simulink model "rfsoc4x2_ospfb_128"  (R2021a)
settings: Solver=VariableStepAuto  StartTime=0.0  StopTime=2048  RelTol=1e-3
undefined symbols (not defined in the file): pfb_coeff_gen_calc
libraries: xbsIndex_r4 x25898, casper_library_delays x113, casper_library_misc x68, xps_library x1
(part 15 of 221)

== system rfsoc4x2_ospfb_128/rfdc ==
  m00_axis_tdata_sim : Inport
  m02_axis_tdata_sim : Inport  Port=2
  m10_axis_tdata_sim : Inport  Port=3
  m12_axis_tdata_sim : Inport  Port=4
  m20_axis_tdata_sim : Inport  Port=5
  m22_axis_tdata_sim : Inport  Port=6
  m30_axis_tdata_sim : Inport  Port=7
  m32_axis_tdata_sim : Inport  Port=8
  rfsoc4x2_ospfb_128_rfdc_m00_axis_tdata : xbsIndex_r4/Gateway In  gui_display_data_type=Fixed-point  arith_type="Signed  (2's comp)"  n_bits=128  bin_pt=0  preci_type=Single  exp_width=8  frac_width=24  rows=1  columns=1  quantization="Round  (unbiased: +/- Inf)"  overflow=Saturate  period=1  UseAsADC=off  ADCChannel='1'  interface=None  automatic_assignment=on  address_offset=hex2dec('00')  intf_name=''  intf_description=''  default_value=0  timing_constraint=None  locs_specified=off  LOCs={}  io_standard={}  inherit_from_input=off  hdl_port=on  dbl_ovrd=off  block_type=gatewayin
  rfsoc4x2_ospfb_128_rfdc_m02_axis_tdata : xbsIndex_r4/Gateway In  gui_display_data_type=Fixed-point  arith_type="Signed  (2's comp)"  n_bits=128  bin_pt=0  preci_type=Single  exp_width=8  frac_width=24  rows=1  columns=1  quantization="Round  (unbiased: +/- Inf)"  overflow=Saturate  period=1  UseAsADC=off  ADCChannel='1'  interface=None  automatic_assignment=on  address_offset=hex2dec('00')  intf_name=''  intf_description=''  default_value=0  timing_constraint=None  locs_specified=off  LOCs={}  io_standard={}  inherit_from_input=off  hdl_port=on  dbl_ovrd=off  block_type=gatewayin
  rfsoc4x2_ospfb_128_rfdc_m10_axis_tdata : xbsIndex_r4/Gateway In  gui_display_data_type=Fixed-point  arith_type="Signed  (2's comp)"  n_bits=128  bin_pt=0  preci_type=Single  exp_width=8  frac_width=24  rows=1  columns=1  quantization="Round  (unbiased: +/- Inf)"  overflow=Saturate  period=1  UseAsADC=off  ADCChannel='1'  interface=None  automatic_assignment=on  address_offset=hex2dec('00')  intf_name=''  intf_description=''  default_value=0  timing_constraint=None  locs_specified=off  LOCs={}  io_standard={}  inherit_from_input=off  hdl_port=on  dbl_ovrd=off  block_type=gatewayin
  rfsoc4x2_ospfb_128_rfdc_m12_axis_tdata : xbsIndex_r4/Gateway In  gui_display_data_type=Fixed-point  arith_type="Signed  (2's comp)"  n_bits=128  bin_pt=0  preci_type=Single  exp_width=8  frac_width=24  rows=1  columns=1  quantization="Round  (unbiased: +/- Inf)"  overflow=Saturate  period=1  UseAsADC=off  ADCChannel='1'  interface=None  automatic_assignment=on  address_offset=hex2dec('00')  intf_name=''  intf_description=''  default_value=0  timing_constraint=None  locs_specified=off  LOCs={}  io_standard={}  inherit_from_input=off  hdl_port=on  dbl_ovrd=off  block_type=gatewayin
  rfsoc4x2_ospfb_128_rfdc_m20_axis_tdata : xbsIndex_r4/Gateway In  gui_display_data_type=Fixed-point  arith_type="Signed  (2's comp)"  n_bits=128  bin_pt=0  preci_type=Single  exp_width=8  frac_width=24  rows=1  columns=1  quantization="Round  (unbiased: +/- Inf)"  overflow=Saturate  period=1  UseAsADC=off  ADCChannel='1'  interface=None  automatic_assignment=on  address_offset=hex2dec('00')  intf_name=''  intf_description=''  default_value=0  timing_constraint=None  locs_specified=off  LOCs={}  io_standard={}  inherit_from_input=off  hdl_port=on  dbl_ovrd=off  block_type=gatewayin
  rfsoc4x2_ospfb_128_rfdc_m22_axis_tdata : xbsIndex_r4/Gateway In  gui_display_data_type=Fixed-point  arith_type="Signed  (2's comp)"  n_bits=128  bin_pt=0  preci_type=Single  exp_width=8  frac_width=24  rows=1  columns=1  quantization="Round  (unbiased: +/- Inf)"  overflow=Saturate  period=1  UseAsADC=off  ADCChannel='1'  interface=None  automatic_assignment=on  address_offset=hex2dec('00')  intf_name=''  intf_description=''  default_value=0  timing_constraint=None  locs_specified=off  LOCs={}  io_standard={}  inherit_from_input=off  hdl_port=on  dbl_ovrd=off  block_type=gatewayin
  rfsoc4x2_ospfb_128_rfdc_m30_axis_tdata : xbsIndex_r4/Gateway In  gui_display_data_type=Fixed-point  arith_type="Signed  (2's comp)"  n_bits=128  bin_pt=0  preci_type=Single  exp_width=8  frac_width=24  rows=1  columns=1  quantization="Round  (unbiased: +/- Inf)"  overflow=Saturate  period=1  UseAsADC=off  ADCChannel='1'  interface=None  automatic_assignment=on  address_offset=hex2dec('00')  intf_name=''  intf_description=''  default_value=0  timing_constraint=None  locs_specified=off  LOCs={}  io_standard={}  inherit_from_input=off  hdl_port=on  dbl_ovrd=off  block_type=gatewayin
  rfsoc4x2_ospfb_128_rfdc_m32_axis_tdata : xbsIndex_r4/Gateway In  gui_display_data_type=Fixed-point  arith_type="Signed  (2's comp)"  n_bits=128  bin_pt=0  preci_type=Single  exp_width=8  frac_width=24  rows=1  columns=1  quantization="Round  (unbiased: +/- Inf)"  overflow=Saturate  period=1  UseAsADC=off  ADCChannel='1'  interface=None  automatic_assignment=on  address_offset=hex2dec('00')  intf_name=''  intf_description=''  default_value=0  timing_constraint=None  locs_specified=off  LOCs={}  io_standard={}  inherit_from_input=off  hdl_port=on  dbl_ovrd=off  block_type=gatewayin
  m00_axis_tdata : Outport
  m02_axis_tdata : Outport  Port=2
  m10_axis_tdata : Outport  Port=3
  m12_axis_tdata : Outport  Port=4
  m20_axis_tdata : Outport  Port=5
  m22_axis_tdata : Outport  Port=6
  m30_axis_tdata : Outport  Port=7
  m32_axis_tdata : Outport  Port=8
  wires:
  m00_axis_tdata_sim/1 -> rfsoc4x2_ospfb_128_rfdc_m00_axis_tdata/1
  rfsoc4x2_ospfb_128_rfdc_m00_axis_tdata/1 -> m00_axis_tdata/1  "m00_axis_tdata"
  m02_axis_tdata_sim/1 -> rfsoc4x2_ospfb_128_rfdc_m02_axis_tdata/1
  rfsoc4x2_ospfb_128_rfdc_m02_axis_tdata/1 -> m02_axis_tdata/1  "m02_axis_tdata"
  m10_axis_tdata_sim/1 -> rfsoc4x2_ospfb_128_rfdc_m10_axis_tdata/1
  rfsoc4x2_ospfb_128_rfdc_m10_axis_tdata/1 -> m10_axis_tdata/1  "m10_axis_tdata"
  m12_axis_tdata_sim/1 -> rfsoc4x2_ospfb_128_rfdc_m12_axis_tdata/1
  rfsoc4x2_ospfb_128_rfdc_m12_axis_tdata/1 -> m12_axis_tdata/1  "m12_axis_tdata"
  m20_axis_tdata_sim/1 -> rfsoc4x2_ospfb_128_rfdc_m20_axis_tdata/1
  rfsoc4x2_ospfb_128_rfdc_m20_axis_tdata/1 -> m20_axis_tdata/1  "m20_axis_tdata"
  m22_axis_tdata_sim/1 -> rfsoc4x2_ospfb_128_rfdc_m22_axis_tdata/1
  rfsoc4x2_ospfb_128_rfdc_m22_axis_tdata/1 -> m22_axis_tdata/1  "m22_axis_tdata"
  m30_axis_tdata_sim/1 -> rfsoc4x2_ospfb_128_rfdc_m30_axis_tdata/1
  rfsoc4x2_ospfb_128_rfdc_m30_axis_tdata/1 -> m30_axis_tdata/1  "m30_axis_tdata"
  m32_axis_tdata_sim/1 -> rfsoc4x2_ospfb_128_rfdc_m32_axis_tdata/1
  rfsoc4x2_ospfb_128_rfdc_m32_axis_tdata/1 -> m32_axis_tdata/1  "m32_axis_tdata"

== system rfsoc4x2_ospfb_128/simple_bram_vacc10 ==
  new_acc : Inport
  din : Inport  Port=2
  Adder : xbsIndex_r4/AddSub  mode=Addition  use_carryin=off  use_carryout=off  en=off  latency=2  precision=User Defined  arith_type=Unsigned  n_bits=n_bits  bin_pt=bin_pt  quantization=Truncate  overflow=Wrap  use_behavioral_HDL=on  hw_selection=Fabric  pipelined=off  use_rpm=on  dbl_ovrd=off  block_type=addsub
      settings: xl_area=[0, 0, 0, 0, 0, 0, 0]  block_version=10.1.3
  Constant : xbsIndex_r4/Constant  const=0  gui_display_data_type=Fixed-point  arith_type=Unsigned  n_bits=n_bits  bin_pt=bin_pt  preci_type=Single  exp_width=8  frac_width=24  explicit_period=on  period=1  equ=P=C  opselect=C  inp2=PCIN>>17  opr=+  inp1=P  carry=CIN  dbl_ovrd=off  block_type=constant
  Mux : xbsIndex_r4/Mux  inputs=2  en=off  latency=0  precision=Full  arith_type="Signed  (2's comp)"  n_bits=8  bin_pt=2  quantization=Truncate  overflow=Wrap  dbl_ovrd=off  block_type=mux
      settings: xl_area=[0, 0, 0, 0, 0, 0, 0]
  delay_bram : Subsystem  mask(delay_bram){DelayLen=vec_len - 2, bram_latency=2}
      mask prompts: DelayLen "Delay By:"; bram_latency "BRAM Latency"
      mask help: A delay block that uses BRAM for its storage.
      mask init:
      | if (DelayLen <= bram_latency)
      | 	error('delay value must be greater than BRAM Latency');
      | end
      | BitWidth = max(ceil(log2(DelayLen)), 2);
      mask Help: eval('xlWeb(''http://casper.berkeley.edu/wiki/Delay_bram'')')
  pulse_ext : Subsystem  mask(pulse_ext){pulse_len=vec_len}
      mask prompts: pulse_len "Length of Pulse"
      mask help:
      | Extends a boolean signal to be high for the specified number of clocks after
      | the last high input.
      mask init:
      | bits = ceil(log2(pulse_len+1));
      mask Help: eval('xlWeb(''http://casper.berkeley.edu/wiki/Pulse_ext'')')
  dout : Outport  VectorParamsAs1DForOutWhenUnconnected=off
  valid : Outport  Port=2  VectorParamsAs1DForOutWhenUnconnected=off
  wires:
  Adder/1 -> delay_bram/1(In1)
  delay_bram/1(Out1) -> dout/1, Mux/2
  new_acc/1 -> pulse_ext/1(in)
  din/1 -> Adder/1
  pulse_ext/1(out) -> valid/1, Mux/1
  Mux/1 -> Adder/2
  Constant/1 -> Mux/3

== system rfsoc4x2_ospfb_128/simple_bram_vacc11 ==
  new_acc : Inport
  din : Inport  Port=2
  Adder : xbsIndex_r4/AddSub  mode=Addition  use_carryin=off  use_carryout=off  en=off  latency=2  precision=User Defined  arith_type=Unsigned  n_bits=n_bits  bin_pt=bin_pt  quantization=Truncate  overflow=Wrap  use_behavioral_HDL=on  hw_selection=Fabric  pipelined=off  use_rpm=on  dbl_ovrd=off  block_type=addsub
      settings: xl_area=[0, 0, 0, 0, 0, 0, 0]  block_version=10.1.3
  Constant : xbsIndex_r4/Constant  const=0  gui_display_data_type=Fixed-point  arith_type=Unsigned  n_bits=n_bits  bin_pt=bin_pt  preci_type=Single  exp_width=8  frac_width=24  explicit_period=on  period=1  equ=P=C  opselect=C  inp2=PCIN>>17  opr=+  inp1=P  carry=CIN  dbl_ovrd=off  block_type=constant
  Mux : xbsIndex_r4/Mux  inputs=2  en=off  latency=0  precision=Full  arith_type="Signed  (2's comp)"  n_bits=8  bin_pt=2  quantization=Truncate  overflow=Wrap  dbl_ovrd=off  block_type=mux
      settings: xl_area=[0, 0, 0, 0, 0, 0, 0]
  delay_bram : Subsystem  mask(delay_bram){DelayLen=vec_len - 2, bram_latency=2}
      mask prompts: DelayLen "Delay By:"; bram_latency "BRAM Latency"
      mask help: A delay block that uses BRAM for its storage.
      mask init:
      | if (DelayLen <= bram_latency)
      | 	error('delay value must be greater than BRAM Latency');
      | end
      | BitWidth = max(ceil(log2(DelayLen)), 2);
      mask Help: eval('xlWeb(''http://casper.berkeley.edu/wiki/Delay_bram'')')
  pulse_ext : Subsystem  mask(pulse_ext){pulse_len=vec_len}
      mask prompts: pulse_len "Length of Pulse"
      mask help:
      | Extends a boolean signal to be high for the specified number of clocks after
      | the last high input.
      mask init:
      | bits = ceil(log2(pulse_len+1));
      mask Help: eval('xlWeb(''http://casper.berkeley.edu/wiki/Pulse_ext'')')
  dout : Outport  VectorParamsAs1DForOutWhenUnconnected=off
  valid : Outport  Port=2  VectorParamsAs1DForOutWhenUnconnected=off
  wires:
  Adder/1 -> delay_bram/1(In1)
  delay_bram/1(Out1) -> dout/1, Mux/2
  new_acc/1 -> pulse_ext/1(in)
  din/1 -> Adder/1
  pulse_ext/1(out) -> valid/1, Mux/1
  Mux/1 -> Adder/2
  Constant/1 -> Mux/3

== system rfsoc4x2_ospfb_128/simple_bram_vacc12 ==
  new_acc : Inport
  din : Inport  Port=2
  Adder : xbsIndex_r4/AddSub  mode=Addition  use_carryin=off  use_carryout=off  en=off  latency=2  precision=User Defined  arith_type=Unsigned  n_bits=n_bits  bin_pt=bin_pt  quantization=Truncate  overflow=Wrap  use_behavioral_HDL=on  hw_selection=Fabric  pipelined=off  use_rpm=on  dbl_ovrd=off  block_type=addsub
      settings: xl_area=[0, 0, 0, 0, 0, 0, 0]  block_version=10.1.3
  Constant : xbsIndex_r4/Constant  const=0  gui_display_data_type=Fixed-point  arith_type=Unsigned  n_bits=n_bits  bin_pt=bin_pt  preci_type=Single  exp_width=8  frac_width=24  explicit_period=on  period=1  equ=P=C  opselect=C  inp2=PCIN>>17  opr=+  inp1=P  carry=CIN  dbl_ovrd=off  block_type=constant
  Mux : xbsIndex_r4/Mux  inputs=2  en=off  latency=0  precision=Full  arith_type="Signed  (2's comp)"  n_bits=8  bin_pt=2  quantization=Truncate  overflow=Wrap  dbl_ovrd=off  block_type=mux
      settings: xl_area=[0, 0, 0, 0, 0, 0, 0]
  delay_bram : Subsystem  mask(delay_bram){DelayLen=vec_len - 2, bram_latency=2}
      mask prompts: DelayLen "Delay By:"; bram_latency "BRAM Latency"
      mask help: A delay block that uses BRAM for its storage.
      mask init:
      | if (DelayLen <= bram_latency)
      | 	error('delay value must be greater than BRAM Latency');
      | end
      | BitWidth = max(ceil(log2(DelayLen)), 2);
      mask Help: eval('xlWeb(''http://casper.berkeley.edu/wiki/Delay_bram'')')
  pulse_ext : Subsystem  mask(pulse_ext){pulse_len=vec_len}
      mask prompts: pulse_len "Length of Pulse"
      mask help:
      | Extends a boolean signal to be high for the specified number of clocks after
      | the last high input.
      mask init:
      | bits = ceil(log2(pulse_len+1));
      mask Help: eval('xlWeb(''http://casper.berkeley.edu/wiki/Pulse_ext'')')
  dout : Outport  VectorParamsAs1DForOutWhenUnconnected=off
  valid : Outport  Port=2  VectorParamsAs1DForOutWhenUnconnected=off
  wires:
  Adder/1 -> delay_bram/1(In1)
  delay_bram/1(Out1) -> dout/1, Mux/2
  new_acc/1 -> pulse_ext/1(in)
  din/1 -> Adder/1
  pulse_ext/1(out) -> valid/1, Mux/1
  Mux/1 -> Adder/2
  Constant/1 -> Mux/3

== system rfsoc4x2_ospfb_128/simple_bram_vacc13 ==
  new_acc : Inport
  din : Inport  Port=2
  Adder : xbsIndex_r4/AddSub  mode=Addition  use_carryin=off  use_carryout=off  en=off  latency=2  precision=User Defined  arith_type=Unsigned  n_bits=n_bits  bin_pt=bin_pt  quantization=Truncate  overflow=Wrap  use_behavioral_HDL=on  hw_selection=Fabric  pipelined=off  use_rpm=on  dbl_ovrd=off  block_type=addsub
      settings: xl_area=[0, 0, 0, 0, 0, 0, 0]  block_version=10.1.3
  Constant : xbsIndex_r4/Constant  const=0  gui_display_data_type=Fixed-point  arith_type=Unsigned  n_bits=n_bits  bin_pt=bin_pt  preci_type=Single  exp_width=8  frac_width=24  explicit_period=on  period=1  equ=P=C  opselect=C  inp2=PCIN>>17  opr=+  inp1=P  carry=CIN  dbl_ovrd=off  block_type=constant
  Mux : xbsIndex_r4/Mux  inputs=2  en=off  latency=0  precision=Full  arith_type="Signed  (2's comp)"  n_bits=8  bin_pt=2  quantization=Truncate  overflow=Wrap  dbl_ovrd=off  block_type=mux
      settings: xl_area=[0, 0, 0, 0, 0, 0, 0]
  delay_bram : Subsystem  mask(delay_bram){DelayLen=vec_len - 2, bram_latency=2}
      mask prompts: DelayLen "Delay By:"; bram_latency "BRAM Latency"
      mask help: A delay block that uses BRAM for its storage.
      mask init:
      | if (DelayLen <= bram_latency)
      | 	error('delay value must be greater than BRAM Latency');
      | end
      | BitWidth = max(ceil(log2(DelayLen)), 2);
      mask Help: eval('xlWeb(''http://casper.berkeley.edu/wiki/Delay_bram'')')
  pulse_ext : Subsystem  mask(pulse_ext){pulse_len=vec_len}
      mask prompts: pulse_len "Length of Pulse"
      mask help:
      | Extends a boolean signal to be high for the specified number of clocks after
      | the last high input.
      mask init:
      | bits = ceil(log2(pulse_len+1));
      mask Help: eval('xlWeb(''http://casper.berkeley.edu/wiki/Pulse_ext'')')
  dout : Outport  VectorParamsAs1DForOutWhenUnconnected=off
  valid : Outport  Port=2  VectorParamsAs1DForOutWhenUnconnected=off
  wires:
  Adder/1 -> delay_bram/1(In1)
  delay_bram/1(Out1) -> dout/1, Mux/2
  new_acc/1 -> pulse_ext/1(in)
  din/1 -> Adder/1
  pulse_ext/1(out) -> valid/1, Mux/1
  Mux/1 -> Adder/2
  Constant/1 -> Mux/3

== system rfsoc4x2_ospfb_128/simple_bram_vacc14 ==
  new_acc : Inport
  din : Inport  Port=2
  Adder : xbsIndex_r4/AddSub  mode=Addition  use_carryin=off  use_carryout=off  en=off  latency=2  precision=User Defined  arith_type=Unsigned  n_bits=n_bits  bin_pt=bin_pt  quantization=Truncate  overflow=Wrap  use_behavioral_HDL=on  hw_selection=Fabric  pipelined=off  use_rpm=on  dbl_ovrd=off  block_type=addsub
      settings: xl_area=[0, 0, 0, 0, 0, 0, 0]  block_version=10.1.3
  Constant : xbsIndex_r4/Constant  const=0  gui_display_data_type=Fixed-point  arith_type=Unsigned  n_bits=n_bits  bin_pt=bin_pt  preci_type=Single  exp_width=8  frac_width=24  explicit_period=on  period=1  equ=P=C  opselect=C  inp2=PCIN>>17  opr=+  inp1=P  carry=CIN  dbl_ovrd=off  block_type=constant
  Gateway Out5 : xbsIndex_r4/Gateway Out  inherit_from_input=off  hdl_port=on  rows=1  columns=1  UseAsDAC=off  DACChannel='1'  interface=None  automatic_assignment=on  address_offset=hex2dec('00')  intf_name=''  intf_description=''  timing_constraint=None  locs_specified=off  LOCs={}  io_standard={}  block_type=gatewayout
  Mux : xbsIndex_r4/Mux  inputs=2  en=off  latency=0  precision=Full  arith_type="Signed  (2's comp)"  n_bits=8  bin_pt=2  quantization=Truncate  overflow=Wrap  dbl_ovrd=off  block_type=mux
      settings: xl_area=[0, 0, 0, 0, 0, 0, 0]
  Scope23 : Scope
  delay_bram : Subsystem  mask(delay_bram){DelayLen=vec_len - 2, bram_latency=2}
      mask prompts: DelayLen "Delay By:"; bram_latency "BRAM Latency"
      mask help: A delay block that uses BRAM for its storage.
      mask init:
      | if (DelayLen <= bram_latency)
      | 	error('delay value must be greater than BRAM Latency');
      | end
      | BitWidth = max(ceil(log2(DelayLen)), 2);
      mask Help: eval('xlWeb(''http://casper.berkeley.edu/wiki/Delay_bram'')')
  pulse_ext : Subsystem  mask(pulse_ext){pulse_len=vec_len}
      mask prompts: pulse_len "Length of Pulse"
      mask help:
      | Extends a boolean signal to be high for the specified number of clocks after
      | the last high input.
      mask init:
      | bits = ceil(log2(pulse_len+1));
      mask Help: eval('xlWeb(''http://casper.berkeley.edu/wiki/Pulse_ext'')')
  dout : Outport  VectorParamsAs1DForOutWhenUnconnected=off
  valid : Outport  Port=2  VectorParamsAs1DForOutWhenUnconnected=off
  wires:
  Adder/1 -> delay_bram/1(In1)
  delay_bram/1(Out1) -> dout/1, Mux/2
  new_acc/1 -> pulse_ext/1(in)
  din/1 -> Adder/1
  pulse_ext/1(out) -> Gateway Out5/1, valid/1, Mux/1
  Mux/1 -> Adder/2
  Constant/1 -> Mux/3
  Gateway Out5/1 -> Scope23/1

== system rfsoc4x2_ospfb_128/simple_bram_vacc15 ==
  new_acc : Inport
  din : Inport  Port=2
  Adder : xbsIndex_r4/AddSub  mode=Addition  use_carryin=off  use_carryout=off  en=off  latency=2  precision=User Defined  arith_type=Unsigned  n_bits=n_bits  bin_pt=bin_pt  quantization=Truncate  overflow=Wrap  use_behavioral_HDL=on  hw_selection=Fabric  pipelined=off  use_rpm=on  dbl_ovrd=off  block_type=addsub
      settings: xl_area=[0, 0, 0, 0, 0, 0, 0]  block_version=10.1.3
  Constant : xbsIndex_r4/Constant  const=0  gui_display_data_type=Fixed-point  arith_type=Unsigned  n_bits=n_bits  bin_pt=bin_pt  preci_type=Single  exp_width=8  frac_width=24  explicit_period=on  period=1  equ=P=C  opselect=C  inp2=PCIN>>17  opr=+  inp1=P  carry=CIN  dbl_ovrd=off  block_type=constant
  Mux : xbsIndex_r4/Mux  inputs=2  en=off  latency=0  precision=Full  arith_type="Signed  (2's comp)"  n_bits=8  bin_pt=2  quantization=Truncate  overflow=Wrap  dbl_ovrd=off  block_type=mux
      settings: xl_area=[0, 0, 0, 0, 0, 0, 0]
  delay_bram : Subsystem  mask(delay_bram){DelayLen=vec_len - 2, bram_latency=2}
      mask prompts: DelayLen "Delay By:"; bram_latency "BRAM Latency"
      mask help: A delay block that uses BRAM for its storage.
      mask init:
      | if (DelayLen <= bram_latency)
      | 	error('delay value must be greater than BRAM Latency');
      | end
      | BitWidth = max(ceil(log2(DelayLen)), 2);
      mask Help: eval('xlWeb(''http://casper.berkeley.edu/wiki/Delay_bram'')')
  pulse_ext : Subsystem  mask(pulse_ext){pulse_len=vec_len}
      mask prompts: pulse_len "Length of Pulse"
      mask help:
      | Extends a boolean signal to be high for the specified number of clocks after
      | the last high input.
      mask init:
      | bits = ceil(log2(pulse_len+1));
      mask Help: eval('xlWeb(''http://casper.berkeley.edu/wiki/Pulse_ext'')')
  dout : Outport  VectorParamsAs1DForOutWhenUnconnected=off
  valid : Outport  Port=2  VectorParamsAs1DForOutWhenUnconnected=off
  wires:
  Adder/1 -> delay_bram/1(In1)
  delay_bram/1(Out1) -> dout/1, Mux/2
  new_acc/1 -> pulse_ext/1(in)
  din/1 -> Adder/1
  pulse_ext/1(out) -> valid/1, Mux/1
  Mux/1 -> Adder/2
  Constant/1 -> Mux/3

== system rfsoc4x2_ospfb_128/simple_bram_vacc8 ==
  new_acc : Inport
  din : Inport  Port=2
  Adder : xbsIndex_r4/AddSub  mode=Addition  use_carryin=off  use_carryout=off  en=off  latency=2  precision=User Defined  arith_type=Unsigned  n_bits=n_bits  bin_pt=bin_pt  quantization=Truncate  overflow=Wrap  use_behavioral_HDL=on  hw_selection=Fabric  pipelined=off  use_rpm=on  dbl_ovrd=off  block_type=addsub
      settings: xl_area=[0, 0, 0, 0, 0, 0, 0]  block_version=10.1.3
  Constant : xbsIndex_r4/Constant  const=0  gui_display_data_type=Fixed-point  arith_type=Unsigned  n_bits=n_bits  bin_pt=bin_pt  preci_type=Single  exp_width=8  frac_width=24  explicit_period=on  period=1  equ=P=C  opselect=C  inp2=PCIN>>17  opr=+  inp1=P  carry=CIN  dbl_ovrd=off  block_type=constant
  Gateway Out5 : xbsIndex_r4/Gateway Out  inherit_from_input=off  hdl_port=on  rows=1  columns=1  UseAsDAC=off  DACChannel='1'  interface=None  automatic_assignment=on  address_offset=hex2dec('00')  intf_name=''  intf_description=''  timing_constraint=None  locs_specified=off  LOCs={}  io_standard={}  block_type=gatewayout
  Mux : xbsIndex_r4/Mux  inputs=2  en=off  latency=0  precision=Full  arith_type="Signed  (2's comp)"  n_bits=8  bin_pt=2  quantization=Truncate  overflow=Wrap  dbl_ovrd=off  block_type=mux
      settings: xl_area=[0, 0, 0, 0, 0, 0, 0]
  Scope23 : Scope
  delay_bram : Subsystem  mask(delay_bram){DelayLen=vec_len - 2, bram_latency=2}
      mask prompts: DelayLen "Delay By:"; bram_latency "BRAM Latency"
      mask help: A delay block that uses BRAM for its storage.
      mask init:
      | if (DelayLen <= bram_latency)
      | 	error('delay value must be greater than BRAM Latency');
      | end
      | BitWidth = max(ceil(log2(DelayLen)), 2);
      mask Help: eval('xlWeb(''http://casper.berkeley.edu/wiki/Delay_bram'')')
  pulse_ext : Subsystem  mask(pulse_ext){pulse_len=vec_len}
      mask prompts: pulse_len "Length of Pulse"
      mask help:
      | Extends a boolean signal to be high for the specified number of clocks after
      | the last high input.
      mask init:
      | bits = ceil(log2(pulse_len+1));
      mask Help: eval('xlWeb(''http://casper.berkeley.edu/wiki/Pulse_ext'')')
  dout : Outport  VectorParamsAs1DForOutWhenUnconnected=off
  valid : Outport  Port=2  VectorParamsAs1DForOutWhenUnconnected=off
  wires:
  Adder/1 -> delay_bram/1(In1)
  delay_bram/1(Out1) -> dout/1, Mux/2
  new_acc/1 -> pulse_ext/1(in)
  din/1 -> Adder/1
  pulse_ext/1(out) -> Gateway Out5/1, valid/1, Mux/1
  Mux/1 -> Adder/2
  Constant/1 -> Mux/3
  Gateway Out5/1 -> Scope23/1

== system rfsoc4x2_ospfb_128/simple_bram_vacc9 ==
  new_acc : Inport
  din : Inport  Port=2
  Adder : xbsIndex_r4/AddSub  mode=Addition  use_carryin=off  use_carryout=off  en=off  latency=2  precision=User Defined  arith_type=Unsigned  n_bits=n_bits  bin_pt=bin_pt  quantization=Truncate  overflow=Wrap  use_behavioral_HDL=on  hw_selection=Fabric  pipelined=off  use_rpm=on  dbl_ovrd=off  block_type=addsub
      settings: xl_area=[0, 0, 0, 0, 0, 0, 0]  block_version=10.1.3
  Constant : xbsIndex_r4/Constant  const=0  gui_display_data_type=Fixed-point  arith_type=Unsigned  n_bits=n_bits  bin_pt=bin_pt  preci_type=Single  exp_width=8  frac_width=24  explicit_period=on  period=1  equ=P=C  opselect=C  inp2=PCIN>>17  opr=+  inp1=P  carry=CIN  dbl_ovrd=off  block_type=constant
  Mux : xbsIndex_r4/Mux  inputs=2  en=off  latency=0  precision=Full  arith_type="Signed  (2's comp)"  n_bits=8  bin_pt=2  quantization=Truncate  overflow=Wrap  dbl_ovrd=off  block_type=mux
      settings: xl_area=[0, 0, 0, 0, 0, 0, 0]
  delay_bram : Subsystem  mask(delay_bram){DelayLen=vec_len - 2, bram_latency=2}
      mask prompts: DelayLen "Delay By:"; bram_latency "BRAM Latency"
      mask help: A delay block that uses BRAM for its storage.
      mask init:
      | if (DelayLen <= bram_latency)
      | 	error('delay value must be greater than BRAM Latency');
      | end
      | BitWidth = max(ceil(log2(DelayLen)), 2);
      mask Help: eval('xlWeb(''http://casper.berkeley.edu/wiki/Delay_bram'')')
  pulse_ext : Subsystem  mask(pulse_ext){pulse_len=vec_len}
      mask prompts: pulse_len "Length of Pulse"
      mask help:
      | Extends a boolean signal to be high for the specified number of clocks after
      | the last high input.
      mask init:
      | bits = ceil(log2(pulse_len+1));
      mask Help: eval('xlWeb(''http://casper.berkeley.edu/wiki/Pulse_ext'')')
  dout : Outport  VectorParamsAs1DForOutWhenUnconnected=off
  valid : Outport  Port=2  VectorParamsAs1DForOutWhenUnconnected=off
  wires:
  Adder/1 -> delay_bram/1(In1)
  delay_bram/1(Out1) -> dout/1, Mux/2
  new_acc/1 -> pulse_ext/1(in)
  din/1 -> Adder/1
  pulse_ext/1(out) -> valid/1, Mux/1
  Mux/1 -> Adder/2
  Constant/1 -> Mux/3

== system rfsoc4x2_ospfb_128/sync_cnt ==
  out_reg : Inport
  assert_reg : xbsIndex_r4/Assert  assert_type=on  type_source=Explicitly  gui_display_data_type=Fixed-point  arith_type=Unsigned  n_bits=32  bin_pt=0  preci_type=Single  exp_width=8  frac_width=24  assert_rate=off  rate_source=Explicitly  period=1  output_port=on  block_type=assert
  cast_gw : xbsIndex_r4/Convert  gui_display_data_type=Fixed-point  arith_type=Unsigned  n_bits=32  bin_pt=0  float_type=Single  exp_bits=8  fraction_bits=24  quantization=Truncate  overflow=Wrap  en=off  latency=1  pipeline=off  dbl_ovrd=off  block_type=convert
  io_delay : xbsIndex_r4/Delay  rst=off  infoeditControl=Selection of Reset will increase slice count due to use of real FFs and instead of SRLs  en=off  latency=0  reg_retiming=on  dbl_ovrd=off  block_type=delay
  reint1 : xbsIndex_r4/Reinterpret  force_arith_type=on  arith_type=Unsigned  force_bin_pt=on  bin_pt=0  block_type=reinterpret
  rfsoc4x2_ospfb_128_sync_cnt_user_data_in : xbsIndex_r4/Gateway Out  inherit_from_input=off  hdl_port=on  rows=1  columns=1  UseAsDAC=off  DACChannel='1'  interface=None  automatic_assignment=on  address_offset=hex2dec('00')  intf_name=''  intf_description=''  timing_constraint=None  locs_specified=off  LOCs={}  io_standard={}  block_type=gatewayout
  sim_out : Terminator
  sim_out_reg_gw : xbsIndex_r4/Gateway Out  inherit_from_input=off  hdl_port=off  rows=1  columns=1  UseAsDAC=off  DACChannel='1'  interface=None  automatic_assignment=on  address_offset=hex2dec('00')  intf_name=''  intf_description=''  timing_constraint=None  locs_specified=off  LOCs={}  io_standard={}  block_type=gatewayout
  sim_out_reg_sim_delay : xbsIndex_r4/Delay  rst=off  infoeditControl=Selection of Reset will increase slice count due to use of real FFs and instead of SRLs  en=off  latency=1  reg_retiming=on  dbl_ovrd=off  block_type=delay
  sim_out_reg : Outport  VectorParamsAs1DForOutWhenUnconnected=off
  wires:
  sim_out_reg_sim_delay/1 -> sim_out_reg_gw/1
  sim_out_reg_gw/1 -> sim_out_reg/1
  io_delay/1 -> cast_gw/1
  cast_gw/1 -> rfsoc4x2_ospfb_128_sync_cnt_user_data_in/1
  rfsoc4x2_ospfb_128_sync_cnt_user_data_in/1 -> sim_out/1
  out_reg/1 -> sim_out_reg_sim_delay/1, assert_reg/1
  assert_reg/1 -> reint1/1
  reint1/1 -> io_delay/1

== system rfsoc4x2_ospfb_128/sync_gen ==
  Constant : Constant
  Constant1 : Constant  Value=0
  Constant2 : Constant  Value=0
  Counter3 : xbsIndex_r4/Counter  cnt_type=Free Running  cnt_to=Inf  operation=Up  start_count=0  cnt_by_val=1  arith_type=Unsigned  n_bits=32  bin_pt=0  load_pin=off  rst=on  en=off  explicit_period=off  period=1  use_behavioral_HDL=off  implementation=Fabric  use_rpm=on  dbl_ovrd=off  block_type=counter
      settings: xl_area=[0, 0, 0, 0, 0, 0, 0]
  Logical : xbsIndex_r4/Logical  logical_function=OR  inputs=2  en=off  latency=0  precision=Full  arith_type=Unsigned  n_bits=8  bin_pt=2  align_bp=on  dbl_ovrd=off  block_type=logical
      settings: xl_area=[0, 0, 0, 0, 0, 0, 0]
  Logical1 : xbsIndex_r4/Logical  logical_function=OR  inputs=2  en=off  latency=0  precision=Full  arith_type=Unsigned  n_bits=8  bin_pt=2  align_bp=on  dbl_ovrd=off  block_type=logical
      settings: xl_area=[0, 0, 0, 0, 0, 0, 0]
  Mux : xbsIndex_r4/Mux  inputs=2  en=off  latency=0  precision=Full  arith_type=Unsigned  n_bits=16  bin_pt=14  quantization=Truncate  overflow=Wrap  dbl_ovrd=off  block_type=mux
  Relational : xbsIndex_r4/Relational  mode=a=b  op_type=Bool  en=off  latency=1  dbl_ovrd=off  block_type=relational
      settings: xl_area=[0, 0, 0, 0, 0, 0, 0]  block_version=10.1.3
  Slice1 : xbsIndex_r4/Slice  nbits=1  boolean_output=on  mode=Lower Bit Location + Width  bit1=0  base1=MSB of Input  bit0=0  base0=LSB of Input  dbl_ovrd=off  block_type=slice
      settings: infoedit="Extracts a given range of bits from each input sample and presents it at the output.  The output type is ordinarily unsigned with binary point at zero, but can be Boolean when the slice is one bit wide.<P><P>Hardware notes: In hardware this block costs nothing."  block_version=10.1.3
  Slice2 : xbsIndex_r4/Slice  nbits=1  boolean_output=on  mode=Lower Bit Location + Width  bit1=0  base1=MSB of Input  bit0=0  base0=LSB of Input  dbl_ovrd=off  block_type=slice
      settings: infoedit="Extracts a given range of bits from each input sample and presents it at the output.  The output type is ordinarily unsigned with binary point at zero, but can be Boolean when the slice is one bit wide.<P><P>Hardware notes: In hardware this block costs nothing."  block_version=10.1.3
  posedge1 : Subsystem  AncestorBlock=casper_library_misc/edge_detect  mask(edge_detect){edge=Rising, polarity=Active High, x_in=[0 0.08 0.08 0.16 0.16 0.24 0.24 0.32 0.32 0.4], y_in=[-1 -1  1  1  1  1  1  1  1  1], x_out=[0.6 0.68 0.68 0.76 0.76 0.84 0.84 0.92 0.92 1], y_out=[-1 -1  1  1 -1 -1 -1 -1 -1 -1]}
      mask prompts: edge "Edge Type"; polarity "Output Polarity"; x_in "Input X Positions"; y_in "Input Y Positions"; x_out "Output X Positions"; y_out "Output Y Positions"
      mask help: Output is active for one-cycle after each edge of the specified type (i.e. rising, falling or both).
      mask init: same as rfsoc4x2_ospfb_128/edge_detect1
      settings: AttributesFormatString=|
      | rising edges
      | active high
      mask Help: Output is active for one-cycle after each edge of the specified type (i.e. rising, falling, or both).  Latency is zero.
      mask TypeOptions edge: Rising | Falling | Both
      mask TypeOptions polarity: Active High | Active Low
      mask Display:
      | plot(x_in_num,0.5+y_in_num*0.2);
      | plot(x_out_num,0.5+y_out_num*0.2);
  posedge3 : Subsystem  AncestorBlock=casper_library_misc/edge_detect  mask(edge_detect){edge=Rising, polarity=Active High, x_in=[0 0.08 0.08 0.16 0.16 0.24 0.24 0.32 0.32 0.4], y_in=[-1 -1  1  1  1  1  1  1  1  1], x_out=[0.6 0.68 0.68 0.76 0.76 0.84 0.84 0.92 0.92 1], y_out=[-1 -1  1  1 -1 -1 -1 -1 -1 -1]}
      mask prompts: edge "Edge Type"; polarity "Output Polarity"; x_in "Input X Positions"; y_in "Input Y Positions"; x_out "Output X Positions"; y_out "Output Y Positions"
      mask help: Output is active for one-cycle after each edge of the specified type (i.e. rising, falling or both).
      mask init: same as rfsoc4x2_ospfb_128/edge_detect1
      settings: AttributesFormatString=|
      | rising edges
      | active high
      mask Help: Output is active for one-cycle after each edge of the specified type (i.e. rising, falling, or both).  Latency is zero.
      mask TypeOptions edge: Rising | Falling | Both
      mask TypeOptions polarity: Active High | Active Low
      mask Display:
      | plot(x_in_num,0.5+y_in_num*0.2);
      | plot(x_out_num,0.5+y_out_num*0.2);
  sync : Subsystem  Tag=xps:sw_reg  AncestorBlock=xps_library/Memory/software_register  mask(swreg){io_dir=From Processor, io_delay=0, init_val=0, sample_period=1, names=reg, bitwidths=32, bin_pts=0, arith_types=0, sim_port=on, show_format=on}
      mask prompts: io_dir "I/O direction"; io_delay "I/O delay"; init_val "Initial Value"; sample_period "Sample period"; names "Bitfield names [msb...lsb]"; bitwidths "Bitfield widths"; bin_pts "Bitfield binary pts"; arith_types "Bitfield types, ufix=0, fix=1, bool=2"; sim_port "Provide sim input/output?"; show_format "Print format string?"
      mask help: A 32-bit software-accessible register. Can be divided into bitfields of varying widths and types using the fields in the block mask.
      mask init:
      | swreg_init(gcb)
      settings: AttributesFormatString=1input:uf32.0 = 32 bits
      mask TypeOptions io_dir: To Processor | From Processor
      mask Callback io_dir:
      | mask_enables = get_param(gcb, 'MaskEnables');
      | mask_names = get_param(gcb, 'MaskNames');
      | if strcmp(get_param(gcb, 'io_dir'), 'To Processor'),
      |     mask_enables{ismember(mask_names, 'sample_period')} = 'off';
      | else
      |     mask_enables{ismember(mask_names, 'sample_period')} = 'on';
      | end
      | set_param(gcb, 'MaskEnables', mask_enables);
      mask DialogControl ParameterTabVar0 Prompt: Setup
  sync_period_const : xbsIndex_r4/Constant  const=131070  gui_display_data_type=Fixed-point  arith_type=Signed (2's comp)  n_bits=32  bin_pt=0  preci_type=Single  exp_width=8  frac_width=24  explicit_period=off  period=1  equ=P=C  opselect=C  inp2=PCIN>>17  opr=+  inp1=P  carry=CIN  dbl_ovrd=off  block_type=constant
      settings: block_version=10.1.1
  sync_period_sel : Subsystem  Tag=xps:sw_reg  AncestorBlock=xps_library/Memory/software_register  mask(swreg){io_dir=From Processor, io_delay=0, init_val=0, sample_period=1, names=reg, bitwidths=32, bin_pts=0, arith_types=0, sim_port=on, show_format=on}
      mask prompts: io_dir "I/O direction"; io_delay "I/O delay"; init_val "Initial Value"; sample_period "Sample period"; names "Bitfield names [msb...lsb]"; bitwidths "Bitfield widths"; bin_pts "Bitfield binary pts"; arith_types "Bitfield types, ufix=0, fix=1, bool=2"; sim_port "Provide sim input/output?"; show_format "Print format string?"
      mask help: A 32-bit software-accessible register. Can be divided into bitfields of varying widths and types using the fields in the block mask.
      mask init:
      | swreg_init(gcb)
      settings: AttributesFormatString=1input:uf32.0 = 32 bits
      mask TypeOptions io_dir: To Processor | From Processor
      mask Callback io_dir:
      | mask_enables = get_param(gcb, 'MaskEnables');
      | mask_names = get_param(gcb, 'MaskNames');
      | if strcmp(get_param(gcb, 'io_dir'), 'To Processor'),
      |     mask_enables{ismember(mask_names, 'sample_period')} = 'off';
      | else
      |     mask_enables{ismember(mask_names, 'sample_period')} = 'on';
      | end
      | set_param(gcb, 'MaskEnables', mask_enables);
      mask DialogControl ParameterTabVar0 Prompt: Setup
  sync_period_var : Subsystem  Tag=xps:sw_reg  AncestorBlock=xps_library/Memory/software_register  mask(swreg){io_dir=From Processor, io_delay=0, init_val=0, sample_period=1, names=reg, bitwidths=32, bin_pts=0, arith_types=0, sim_port=on, show_format=on}
      mask prompts: io_dir "I/O direction"; io_delay "I/O delay"; init_val "Initial Value"; sample_period "Sample period"; names "Bitfield names [msb...lsb]"; bitwidths "Bitfield widths"; bin_pts "Bitfield binary pts"; arith_types "Bitfield types, ufix=0, fix=1, bool=2"; sim_port "Provide sim input/output?"; show_format "Print format string?"
      mask help: A 32-bit software-accessible register. Can be divided into bitfields of varying widths and types using the fields in the block mask.
      mask init:
      | swreg_init(gcb)
      settings: AttributesFormatString=1input:uf32.0 = 32 bits
      mask TypeOptions io_dir: To Processor | From Processor
      mask Callback io_dir:
      | mask_enables = get_param(gcb, 'MaskEnables');
      | mask_names = get_param(gcb, 'MaskNames');
      | if strcmp(get_param(gcb, 'io_dir'), 'To Processor'),
      |     mask_enables{ismember(mask_names, 'sample_period')} = 'off';
      | else
      |     mask_enables{ismember(mask_names, 'sample_period')} = 'on';
      | end
      | set_param(gcb, 'MaskEnables', mask_enables);
      mask DialogControl ParameterTabVar0 Prompt: Setup
  sync_out : Outport  VectorParamsAs1DForOutWhenUnconnected=off
  wires:
  sync/1(in_reg) -> posedge3/1(in)
  sync_period_sel/1(in_reg) -> Slice1/1
  sync_period_var/1(in_reg) -> Mux/3
  Constant/1 -> sync/1(sim_1)
  Constant2/1 -> sync_period_var/1(sim_1)
  Constant1/1 -> sync_period_sel/1(sim_1)
  sync_period_const/1 -> Mux/2
  Slice1/1 -> Mux/1
  Mux/1 -> Relational/1
  posedge1/1(out) -> sync_out/1
  Logical/1 -> posedge1/1(in)
  Relational/1 -> Logical1/1, Logical/1
  Counter3/1 -> Relational/2
  Logical1/1 -> Counter3/1
  Slice2/1 -> Logical/2, Logical1/2
  posedge3/1(out) -> Slice2/1

== system rfsoc4x2_ospfb_128/acc_cntrl2/edge_detect ==
  in : Inport
  Delay : xbsIndex_r4/Delay  rst=off  infoeditControl=Selection of Reset will increase slice count due to use of real FFs and instead of SRLs  en=off  latency=1  reg_retiming=off  dbl_ovrd=off  block_type=delay
      settings: xl_area=[0, 0, 0, 0, 0, 0, 0]
  Inverter : xbsIndex_r4/Inverter  en=off  latency=0  dbl_ovrd=off  block_type=inv
      settings: xl_area=[0, 0, 0, 0, 0, 0, 0]
  edge_op : xbsIndex_r4/Logical  logical_function=NOR  inputs=2  en=off  latency=0  precision=Full  arith_type=Unsigned  n_bits=8  bin_pt=2  align_bp=on  dbl_ovrd=off  block_type=logical
      settings: xl_area=[0, 0, 0, 0, 0, 0, 0]
  out : Outport  VectorParamsAs1DForOutWhenUnconnected=off
  wires:
  Inverter/1 -> edge_op/1
  edge_op/1 -> out/1
  in/1 -> Inverter/1, Delay/1
  Delay/1 -> edge_op/2

== system rfsoc4x2_ospfb_128/acc_cntrl2/pipeline15 ==
  d : Inport
  Register0 : xbsIndex_r4/Register  init=0  rst=off  en=off  dbl_ovrd=off  block_type=register
      settings: block_version=11.4
  q : Outport  VectorParamsAs1DForOutWhenUnconnected=off
  wires:
  d/1 -> Register0/1
  Register0/1 -> q/1

== system rfsoc4x2_ospfb_128/fft1/fft_biplex ==
  sync : Inport
  shift : Inport  Port=2
  pol00_in : Inport  Port=3
  pol01_in : Inport  Port=4
  pol02_in : Inport  Port=5
  pol03_in : Inport  Port=6
  pol04_in : Inport  Port=7
  pol05_in : Inport  Port=8
  pol06_in : Inport  Port=9
  pol07_in : Inport  Port=10
  biplex_core : Subsystem  AncestorBlock=casper_library_ffts/biplex_core  mask(biplex_core){n_inputs=4, FFTSize=6, input_bit_width=18, bin_pt_in=17, coeff_bit_width=18, floating_point=off, float_type=custom, exp_width=8, frac_width=24, add_latency=2, mult_latency=2, bram_latency=2, conv_latency=1, add_pipe_latency=0, mult_pipe_latency=0, quantization=Round  (unbiased: +/- Inf), overflow=Wrap, delays_bit_limit=8, coeffs_bit_limit=9, coeff_sharing=off, coeff_decimation=off, max_fanout=4, mult_spec=[2 2 2 2 2 2], bitgrowth=off, max_bits=19, hardcode_shifts=off, shift_schedule=[1 1 1 1 1 1], dsp48_adders=on, async=off}
      mask prompts: n_inputs "Number inputs (2*?)"; FFTSize "Size of FFT: (2^? pts)"; input_bit_width "Input Bit Width"; bin_pt_in "Input binary point"; coeff_bit_width "Coefficient Bit Width"; floating_point "floating point"; float_type "float type"; exp_width "exponent width"; frac_width "fraction width"; add_latency "Add Latency"; mult_latency "Mult Latency"; bram_latency "BRAM Latency"; conv_latency "Convert latency"; add_pipe_latency "Add Interface Pipeline Latency"; mult_pipe_latency "CMult Pipeline Latency"; quantization "Quantization Behavior"; overflow "Overflow Behavior"; delays_bit_limit "Number bits above which to implent stage's delays in BRAM (2^? bits)"; coeffs_bit_limit "Number bits above which to store stage's coefficients in BRAM (2^? bits)"; coeff_sharing "BRAM sharing in coeff storage"; coeff_decimation "Store a fraction of coeff factors where useful"; max_fanout "Maximum fanout"; mult_spec "Multiplier impl. (0=core, 1=embedded, 2=behavioural) (left=1st stage, or just one value)"; bitgrowth "Bit growth instead of shift"; max_bits "Maximum number of bits"; hardcode_shifts "Hardcode shift schedule"; shift_schedule "Shift schedule"; dsp48_adders "Use DSP48s for adders"; async "Asynchronous operation"
      mask help: FFT internal block.
      mask init:
      | biplex_core_init(gcb, ...
      |     'n_inputs', n_inputs, ...
      |     'FFTSize', FFTSize,...
      |     'input_bit_width', input_bit_width,...
      |     'bin_pt_in', bin_pt_in,...
      |     'coeff_bit_width', coeff_bit_width,...
      |     'floating_point', floating_point, ...
      |     'float_type', float_type, ...
      |     'exp_width', exp_width, ...
      |     'frac_width', frac_width, ...       
      |     'async', async, ...
      |     'add_latency', add_latency,...
      |     'mult_latency', mult_latency,...
      |     'bram_latency', bram_latency,...
      |     'conv_latency', conv_latency, ...
      |     'add_pipe_latency', add_pipe_latency, ...
      |     'mult_pipe_latency', mult_pipe_latency, ...        
      |     'quantization', quantization,...
      |     'overflow', overflow,...
      |     'delays_bit_limit', delays_bit_limit, ...
      |     'coeffs_bit_limit', coeffs_bit_limit, ...
      |     'coeff_sharing', coeff_sharing, ...
      |     'coeff_decimation', coeff_decimation, ...
      |     'max_fanout', max_fanout, ...
      |     'mult_spec', mult_spec, ...
      |     'bitgrowth', bitgrowth, ...
      |     'max_bits', max_bits, ...
      |     'hardcode_shifts', hardcode_shifts, ...
      |     'shift_schedule', shift_schedule, ...
      |     'dsp48_adders', dsp48_adders);
      settings: AttributesFormatString=6 stages
      mask Callback floating_point:
      | onoff = get_param(gcb, 'floating_point');
      | if strcmp(onoff,'on')
      |     enable_fixpt = 'off';
      |     set_param_state(gcb, 'float_type', 'on')
      | 
      |     f_type = get_param(gcb, 'float_type');
      |     if strcmp(f_type,'custom')
      |         set_param_state(gcb, 'exp_width', 'on')
      |         set_param_state(gcb, 'frac_width', 'on')
      |     else
      |         set_param_state(gcb, 'exp_width', 'off')
      |         set_param_state(gcb, 'frac_width', 'off')
      |     end
      | 
      | 
      | else
      |     enable_fixpt = 'on';
      |     set_param_state(gcb, 'float_type', 'off')
      |     set_param_state(gcb, 'exp_width', 'off')
      |     set_param_state(gcb, 'frac_width', 'off')
      | end
      | 
      | set_param_state(gcb, 'input_bit_width', enable_fixpt)
      | set_param_state(gcb, 'bin_pt_in', enable_fixpt)
      | set_param_state(gcb, 'coeff_bit_width', enable_fixpt)
      mask TypeOptions float_type: single | custom
      mask Callback float_type:
      | f_type = get_param(gcb, 'float_type');
      | if strcmp(f_type,'custom')
      |     set_param_state(gcb, 'exp_width', 'on')
      |     set_param_state(gcb, 'frac_width', 'on')
      | else
      |     set_param_state(gcb, 'exp_width', 'off')
      |     set_param_state(gcb, 'frac_width', 'off')
      | end
      mask TypeOptions quantization: Truncate | Round  (unbiased: +/- Inf) | Round  (unbiased: Even Values)
      mask TypeOptions overflow: Wrap | Saturate | Error
      mask Callback hardcode_shifts:
      | hardcode_shifts = get_param(gcb, 'hardcode_shifts');
      | set_param_state(gcb, 'shift_schedule', hardcode_shifts);
      mask Callback dsp48_adders: fft_callback_dsp48_adders(gcb);
      mask DialogControl ParameterTabVar0 Prompt: Basic
      mask DialogControl ParameterTabVar01 Prompt: Latency
      mask DialogControl ParameterTabVar012 Prompt: Implementation
  biplex_cplx_unscrambler : Subsystem  AncestorBlock=casper_library_ffts_internal/biplex_cplx_unscrambler  mask(biplex_cplx_unscrambler){FFTSize=6, bram_latency=2, coeffs_bit_limit=9, async=off}
      mask prompts: FFTSize "Size of FFT: (2^? pnts)"; bram_latency "BRAM Latency"; coeffs_bit_limit "Number bits above which to store stage's coefficients in BRAM (2^? bits)"; async "Asynchronous operation"
      mask init:
      | biplex_cplx_unscrambler_init(gcb, ...
      |     'FFTSize', FFTSize, ...
      |     'bram_latency', bram_latency, ...
      |     'coeffs_bit_limit', coeffs_bit_limit, ...
      |     'async', async);
  even_bussify : Subsystem  AncestorBlock=casper_library_flow_control/bus_create  mask(bus_create){inputNum=4}
      mask prompts: inputNum "Number of inputs:"
      mask init:
      | bus_create_init(gcb,...
      |     'inputNum', inputNum);
  odd_bussify : Subsystem  AncestorBlock=casper_library_flow_control/bus_create  mask(bus_create){inputNum=4}
      mask prompts: inputNum "Number of inputs:"
      mask init:
      | bus_create_init(gcb,...
      |     'inputNum', inputNum);
  pol0_debus : Subsystem  AncestorBlock=casper_library_flow_control/bus_expand  mask(bus_expand){mode=divisions of equal size, outputNum=4, outputWidth=36, outputBinaryPt=0, outputArithmeticType=0, show_format=off, outputToWorkspace=off, variablePrefix=out, outputToModelAsWell=on}
      mask prompts: outputNum "Number of outputs:"; outputWidth "Output width:"; outputBinaryPt "Output binary point position:"; outputArithmeticType "Output arithmetic type (ufix=0, fix=1, bool=2):"; show_format "Print format string?"; outputToWorkspace "Output to workspace?"; variablePrefix "Variable name prefix:"; outputToModelAsWell "Output to model as well?"
      mask help:
      | Expands a 'bus' made using a bus_create or Xilinx
      | concat block.
      | The input will be divided into the specified number
      | of outputs with the specified arithmetic types.
      | Divisions are made from most significant bit.
      mask init: same as rfsoc4x2_ospfb_128/bus_expand
      settings: AttributesFormatString=4 outputs
      mask TypeOptions mode: divisions of equal size | divisions of arbitrary size
      mask Callback mode: %bus_expand_callback();
      mask Callback outputWidth: %bus_expand_callback();
      mask Callback outputToWorkspace: %bus_expand_callback();
  pol1_debus : Subsystem  AncestorBlock=casper_library_flow_control/bus_expand  mask(bus_expand){mode=divisions of equal size, outputNum=4, outputWidth=36, outputBinaryPt=0, outputArithmeticType=0, show_format=off, outputToWorkspace=off, variablePrefix=out, outputToModelAsWell=on}
      mask prompts: outputNum "Number of outputs:"; outputWidth "Output width:"; outputBinaryPt "Output binary point position:"; outputArithmeticType "Output arithmetic type (ufix=0, fix=1, bool=2):"; show_format "Print format string?"; outputToWorkspace "Output to workspace?"; variablePrefix "Variable name prefix:"; outputToModelAsWell "Output to model as well?"
      mask help:
      | Expands a 'bus' made using a bus_create or Xilinx
      | concat block.
      | The input will be divided into the specified number
      | of outputs with the specified arithmetic types.
      | Divisions are made from most significant bit.
      mask init: same as rfsoc4x2_ospfb_128/bus_expand
      settings: AttributesFormatString=4 outputs
      mask TypeOptions mode: divisions of equal size | divisions of arbitrary size
      mask Callback mode: %bus_expand_callback();
      mask Callback outputWidth: %bus_expand_callback();
      mask Callback outputToWorkspace: %bus_expand_callback();
  sync_out : Outport
  pol00_out : Outport  Port=2
  pol01_out : Outport  Port=3
  pol02_out : Outport  Port=4
  pol03_out : Outport  Port=5
  pol04_out : Outport  Port=6
  pol05_out : Outport  Port=7
  pol06_out : Outport  Port=8
  pol07_out : Outport  Port=9
  of : Outport  Port=10
  wires:
  pol00_in/1 -> even_bussify/1(in1)
  pol0_debus/1(msb_out4) -> pol00_out/1
  pol01_in/1 -> odd_bussify/1(in1)
  pol1_debus/1(msb_out4) -> pol01_out/1
  pol02_in/1 -> even_bussify/2(in2)
  pol0_debus/2(out3) -> pol02_out/1
  pol03_in/1 -> odd_bussify/2(in2)
  pol1_debus/2(out3) -> pol03_out/1
  pol04_in/1 -> even_bussify/3(in3)
  pol0_debus/3(out2) -> pol04_out/1
  pol05_in/1 -> odd_bussify/3(in3)
  pol1_debus/3(out2) -> pol05_out/1
  pol06_in/1 -> even_bussify/4(in4)
  pol0_debus/4(lsb_out1) -> pol06_out/1
  pol07_in/1 -> odd_bussify/4(in4)
  pol1_debus/4(lsb_out1) -> pol07_out/1
  sync/1 -> biplex_core/1(sync)
  shift/1 -> biplex_core/2(shift)
  even_bussify/1(bus_out) -> biplex_core/3(pol1)
  odd_bussify/1(bus_out) -> biplex_core/4(pol2)
  biplex_core/1(sync_out) -> biplex_cplx_unscrambler/3(sync)
  biplex_core/2(out1) -> biplex_cplx_unscrambler/1(even)
  biplex_core/3(out2) -> biplex_cplx_unscrambler/2(odd)
  biplex_core/4(of) -> of/1
  biplex_cplx_unscrambler/3(sync_out) -> sync_out/1
  biplex_cplx_unscrambler/1(pol1) -> pol0_debus/1(bus_in)
  biplex_cplx_unscrambler/2(pol2) -> pol1_debus/1(bus_in)
